simulink model "Terasic_Simscape_LQR_2PWM_DISTURBED"  (R2024b)
settings: Solver=VariableStepAuto  StartTime=0.0  StopTime=40  RelTol=1e-3  AbsTol=1e-3  EnableMultiTasking=on
undefined symbols (not defined in the file or in its folder): chassis_mass, dt, gear, joint_friction, K_dlqr, k_t, max_pwm, motor_max_torque, R_int, rotor_inertia, V_nom, wheel_mass, wheel_radius, wheel_track, X, Y, Z
libraries: sm_lib x29, nesl_utility x18, simulink x2
settings Model: Creator=monet  LastModifiedBy=monet
settings SolverCC: AutoScaleAbsTol=off  AlgebraicLoopSolver=TrustRegion  MaxZcPerStep=1
settings DataIOCC: LimitDataPoints=on  MaxDataPoints=10000
settings OptimizationCC: BlockReduction=off  DefaultParameterBehavior=Inlined  BufferReuse=off  ReuseModelBlockBuffer=off  LifeSpan=inf
settings DebuggingCC: UnconnectedInputMsg=warning  UnconnectedOutputMsg=warning  UnconnectedLineMsg=warning  AllowSymbolicDim=off  SubsystemReferenceDiagnosticForUnitTest=warning  SFUnexpectedBacktrackingDiag=warning  SFNoUnconditionalDefaultTransitionDiag=warning  SFExecutionAtInitializationDiag=none  ArithmeticOperatorsInVariantConditions=warning
settings ModelReferenceCC: EnableRefExpFcnMdlSchedulingChecks=on
settings SFSimCC: SimUseLocalCustomCode=off  CustomCodeUndefinedFunction=UseInterfaceOnly
settings RTWCC: RTWUseLocalCustomCode=off  GPUComputeCapability=3.5  DLArmComputeVersion=19.05
settings CodeAppCC: StateflowObjectComments=on
settings GRTTargetCC: TargetLangStandard=C89/C90 (ANSI)
settings ConfigComp: CovMetricSettings=dw  CovSaveCumulativeToWorkspaceVar=on  CovSaveSingleToWorkspaceVar=on  CovExternalEMLEnable=off  CovSFcnEnable=off
settings SimscapeCC: SimscapeLogType=all  SimscapeLogSimulationStatistics=on  SimscapeLogDataHistory=10000
settings ExplorerConfigSet: InternalSimMechanicsExplorerSettings="<ExplorerConfiguration><canonicalview>default</canonicalview><AnimationSetting><BasePlaybackSpeed>1.0</BasePlaybackSpeed><PlaybackSpeedFactor>1.0</PlaybackSpeedFactor></AnimationSetting><TilePanel><TileInfo><Tiles Columns=\"1\" Count=\"1\" Rows=\"1\"><Column Weight=\"1\"/><Row Weight=\"1\"/><Tile Height=\"1\" Width=\"1\" X=\"0\" Y=\"0\"/></Tiles></TileInfo><SceneInfo><SceneViewer><BGColor><R>0.60000002384185791</R><G>0.60000002384185791</G><B>0.60000002384185791</B></BGColor><Camera><DoPerspective>off</DoPerspective><Position><X>0.347323457562067783</X><Y>0.515589851628267981</Y><Z>1.53123320149964282</Z></Position><Center><X>0.0533393895155996889</X><Y>-0.0401565567814901048</Y><Z>0.259834581816526411</Z></Center><Up><X>0.974608991684094539</X><Y>-0.00336145818059463419</Y><Z>-0.22388839614283837</Z></Up><ViewLimDist>1</ViewLimDist><YLim>0.251495735782762964</YLim><XLim>0.488937298095312722</XLim></Camera></SceneViewer></SceneInfo></TilePanel><MechEditorPanel><Cameras/><GfxPanelCameraMap/><VideoCreator><PlaybackSpeedRatio>1.0</PlaybackSpeedRatio><FrameRate>30</FrameRate><VideoFormat>Motion JPEG AVI</VideoFormat><FrameSize>auto</FrameSize></VideoCreator></MechEditorPanel></ExplorerConfiguration>"

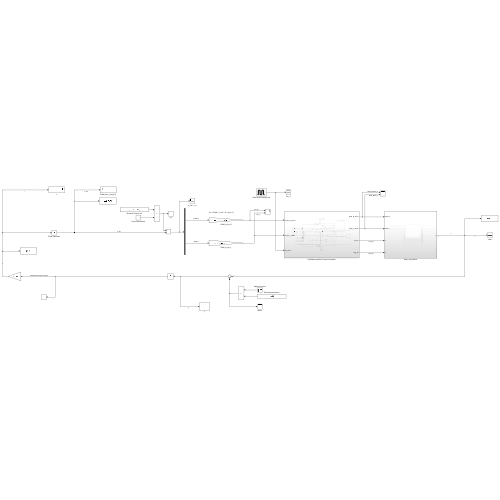
[thumbnail: Simulink's stored preview of the top-level diagram]
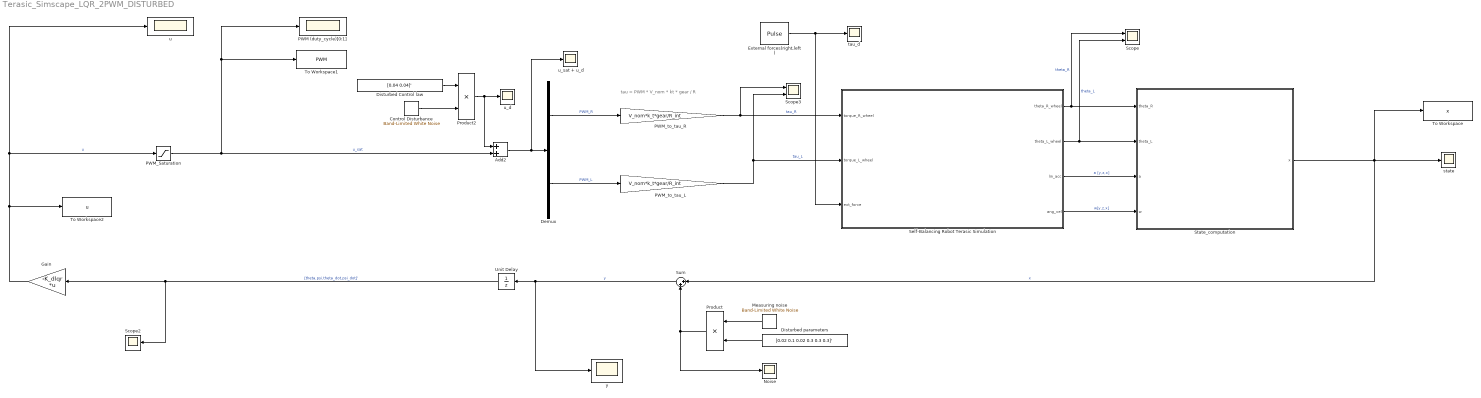
== system Terasic_Simscape_LQR_2PWM_DISTURBED ==
  note: tau = PWM * V_nom * kt * gear / R
  Add2 : Sum
  Control Disturbance : simulink/Sources/Band-Limited White Noise  Cov=[0.001]  Ts=0.1  seed=[23341]
  Demux : Demux  Outputs=2
  Disturbed Control law : Constant  Value=[0.04 0.04]'
  Disturbed parameters : Constant  Value=[0.02 0.1 0.02 0.3 0.3 0.3]'
  External forces(right,left) : DiscretePulseGenerator  PulseType=Time based  Amplitude=0.5  Period=5  PulseWidth=10  PhaseDelay=2
  Gain : Gain  Gain=-K_dlqr  Multiplication=Matrix(K*u)
  Measuring noise : simulink/Sources/Band-Limited White Noise  Cov=[0.001]  Ts=0.1  seed=[23341]
  Noise : Scope
  PWM (duty_cycle)[0:1] : Scope
  PWM_Saturation : Saturate  UpperLimit=max_pwm  LowerLimit=-max_pwm
  PWM_to_tau_L : Gain  Gain=V_nom*k_t*gear/R_int
  PWM_to_tau_R : Gain  Gain=V_nom*k_t*gear/R_int
  Product : Product
  Product2 : Product
  Scope : Scope  NumInputPorts=2
  Scope2 : Scope
  Scope3 : Scope  NumInputPorts=2
  Self-Balancing Robot Terasic Simulation : Subsystem
  State_computation : Subsystem
  Sum : Sum  Inputs=|++
  To Workspace : ToWorkspace  VariableName=x  SaveFormat=Timeseries  SampleTime=-1
  To Workspace1 : ToWorkspace  VariableName=PWM  SaveFormat=Timeseries  SampleTime=-1
  To Workspace2 : ToWorkspace  VariableName=u  SaveFormat=Timeseries  SampleTime=-1
  Unit Delay : UnitDelay  InitialCondition=[0;0;0;0;0;0]  SampleTime=dt  HasFrameUpgradeWarning=on
  state : Scope
  tau_d : Scope
  u : Scope
  u_d : Scope
  u_sat + u_d : Scope
  y : Scope
  wires:
  PWM_to_tau_L/1 -> Self-Balancing Robot Terasic Simulation/2(torque_L_wheel), Scope3/2  "tau_L"
  PWM_to_tau_R/1 -> Self-Balancing Robot Terasic Simulation/1(torque_R_wheel), Scope3/1  "tau_R"
  PWM_Saturation/1 -> To Workspace1/1, PWM (duty_cycle)[0:1]/1, Add2/2  "u_sat"
  Demux/1 -> PWM_to_tau_R/1  "PWM_R"
  Demux/2 -> PWM_to_tau_L/1  "PWM_L"
  Unit Delay/1 -> Scope2/1, Gain/1  "[theta,psi,theta_dot,psi_dot]'"
  Gain/1 -> u/1, PWM_Saturation/1, To Workspace2/1  "u"
  State_computation/1(x) -> Sum/1, To Workspace/1, state/1  "x"
  Self-Balancing Robot Terasic Simulation/2(theta_L_wheel) -> State_computation/2(theta_L), Scope/2  "theta_L"
  Self-Balancing Robot Terasic Simulation/1(theta_R_wheel) -> State_computation/1(theta_R), Scope/1  "theta_R"
  Self-Balancing Robot Terasic Simulation/4(ang_vel) -> State_computation/4(w)  "w[y,z,x]"
  Self-Balancing Robot Terasic Simulation/3(lin_acc) -> State_computation/3(a)  "a [y,z,x]"
  Control Disturbance/1 -> Product2/2
  Product2/1 -> u_d/1, Add2/1
  Disturbed Control law/1 -> Product2/1
  External forces(right,left)/1 -> Self-Balancing Robot Terasic Simulation/3(ext_force), tau_d/1
  Sum/1 -> y/1, Unit Delay/1  "y"
  Measuring noise/1 -> Product/1
  Disturbed parameters/1 -> Product/2
  Product/1 -> Noise/1, Sum/2
  Add2/1 -> u_sat + u_d/1, Demux/1

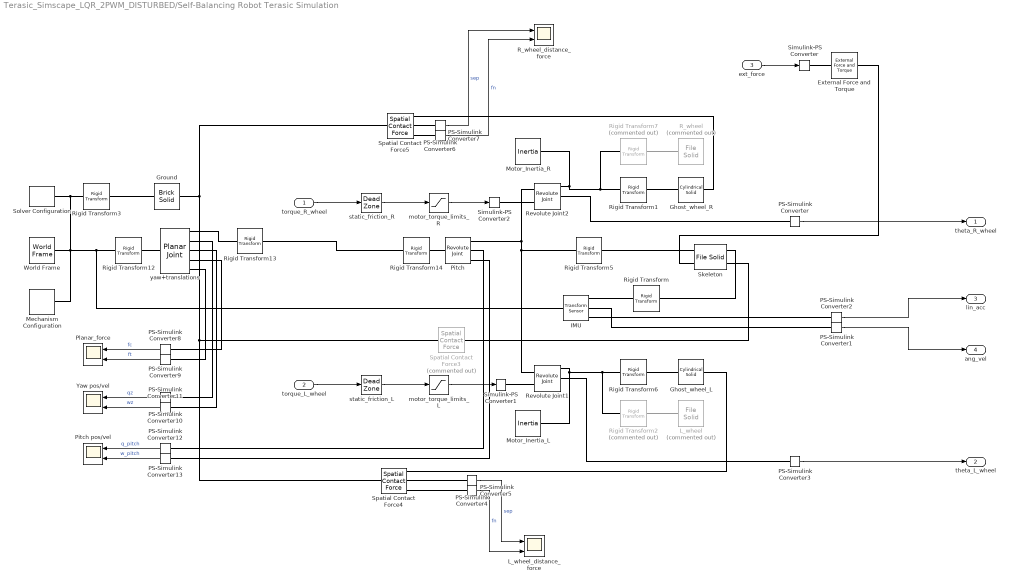
== system Terasic_Simscape_LQR_2PWM_DISTURBED/Self-Balancing Robot Terasic Simulation ==
  torque_R_wheel : Inport
  torque_L_wheel : Inport  Port=2
  ext_force : Inport  Port=3
  External Force and Torque : sm_lib/Forces and Torques/External Force and Torque  EnableForceX=off  EnableForceY=on  EnableForceZ=off  EnableForce=off  ForceResolutionFrame=AttachedFrame  EnableTorqueX=off  EnableTorqueY=off  EnableTorqueZ=off  EnableTorque=off  TorqueResolutionFrame=AttachedFrame
  Ghost_wheel_L : sm_lib/Body Elements/Cylindrical Solid  CylinderRadius=wheel_radius  CylinderRadiusUnits=m  CylinderLength=wheel_thickness  CylinderLengthUnits=m  ExportEntireGeometry=on  InertiaType=CalculateFromGeometry  BasedOnType=Mass  Density=1000  DensityUnits=kg/m^3  Mass=wheel_mass  MassUnits=kg  CenterOfMass=[0 0 0]  CenterOfMassUnits=m  MomentsOfInertia=[1 1 1]  MomentsOfInertiaUnits=kg*m^2  ProductsOfInertia=[0 0 0]  ProductsOfInertiaUnits=kg*m^2  GraphicType=FromGeometry  MarkerShape=Sphere  MarkerSize=10  GraphicVisPropType=SimpleVisualProperties  GraphicDiffuseColor=[1 0 0]  GraphicOpacity=0.1  GraphicSpecularColor=[0.5 0.5 0.5 1.0]  GraphicAmbientColor=[0.15 0.15 0.15 1.0]  GraphicEmissiveColor=[0.0 0.0 0.0 1.0]  GraphicShininess=75  DoExposeReferenceFrame=off  SerializedFrames=<Frames><Frame><Id>Frame1</Id><Value><Name>F1</Name><Origin><Source>ReferenceFrame</Source><FeatureName></FeatureName></Origin><PrimaryAxis><DefinedDirection>+Z</DefinedDirection><Source>ReferenceFrame</Source><SourceDirection>+Z</SourceDirection><FeatureName></FeatureName></PrimaryAxis><SecondaryAxis><DefinedDirection>+X</DefinedDirection><Source>ReferenceFrame</Source><SourceDirection>+X</SourceDirection><FeatureName></FeatureName></SecondaryAxis></Value></Frame></Frames>
  Ghost_wheel_R : sm_lib/Body Elements/Cylindrical Solid  CylinderRadius=wheel_radius  CylinderRadiusUnits=m  CylinderLength=wheel_thickness  CylinderLengthUnits=m  ExportEntireGeometry=on  InertiaType=CalculateFromGeometry  BasedOnType=Mass  Density=1000  DensityUnits=kg/m^3  Mass=wheel_mass  MassUnits=kg  CenterOfMass=[0 0 0]  CenterOfMassUnits=m  MomentsOfInertia=[1 1 1]  MomentsOfInertiaUnits=kg*m^2  ProductsOfInertia=[0 0 0]  ProductsOfInertiaUnits=kg*m^2  GraphicType=FromGeometry  MarkerShape=Sphere  MarkerSize=10  GraphicVisPropType=SimpleVisualProperties  GraphicDiffuseColor=[1 0 0]  GraphicOpacity=0.1  GraphicSpecularColor=[0.5 0.5 0.5 1.0]  GraphicAmbientColor=[0.15 0.15 0.15 1.0]  GraphicEmissiveColor=[0.0 0.0 0.0 1.0]  GraphicShininess=75  DoExposeReferenceFrame=off  SerializedFrames=<Frames><Frame><Id>Frame1</Id><Value><Name>F1</Name><Origin><Source>ReferenceFrame</Source><FeatureName></FeatureName></Origin><PrimaryAxis><DefinedDirection>+Z</DefinedDirection><Source>ReferenceFrame</Source><SourceDirection>+Z</SourceDirection><FeatureName></FeatureName></PrimaryAxis><SecondaryAxis><DefinedDirection>+X</DefinedDirection><Source>ReferenceFrame</Source><SourceDirection>+X</SourceDirection><FeatureName></FeatureName></SecondaryAxis></Value></Frame></Frames>
  Ground : sm_lib/Body Elements/Brick Solid  BrickDimensions=[2 2 0.003]  BrickDimensionsUnits=m  ExportEntireGeometry=on  InertiaType=CalculateFromGeometry  BasedOnType=Density  Density=1000  DensityUnits=kg/m^3  Mass=1  MassUnits=kg  CenterOfMass=[0 0 0]  CenterOfMassUnits=m  MomentsOfInertia=[1 1 1]  MomentsOfInertiaUnits=kg*m^2  ProductsOfInertia=[0 0 0]  ProductsOfInertiaUnits=kg*m^2  GraphicType=FromGeometry  MarkerShape=Sphere  MarkerSize=10  GraphicVisPropType=SimpleVisualProperties  GraphicDiffuseColor=[0.9412 0.9412 0.9412]  GraphicOpacity=1  GraphicSpecularColor=[0.5 0.5 0.5 1.0]  GraphicAmbientColor=[0.15 0.15 0.15 1.0]  GraphicEmissiveColor=[0.0 0.0 0.0 1.0]  GraphicShininess=75  DoExposeReferenceFrame=on  SerializedFrames=<Frames/>
  IMU : sm_lib/Frames and Transforms/Transform Sensor  MeasurementFrame=Follower  RotationSequence=XYX  SenseAngle=off  SenseAxis=off  SenseQ=off  SenseR=off  SenseRotationSequence=off  SenseOmegaX=off  SenseOmegaY=off  SenseOmegaZ=off  SenseOmega=on  SenseQDot=off  SenseRDot=off  SenseRotationSequenceDot=off  SenseAlphaX=off  SenseAlphaY=off  SenseAlphaZ=off  SenseAlpha=off  SenseQDDot=off  SenseRDDot=off  SenseX=off  SenseY=off  SenseZ=off  SenseXYZ=off  SenseRad=off  SenseAzim=off  SenseDist=off  SenseInc=off  SenseXDot=off  SenseYDot=off  SenseZDot=off  SenseXYZDot=off  SenseRadDot=off  SenseAzimDot=off  SenseDistDot=off  SenseIncDot=off  SenseXDDot=off  SenseYDDot=off  SenseZDDot=off  SenseXYZDDot=on  SenseRadDDot=off  SenseAzimDDot=off  SenseDistDDot=off  SenseIncDDot=off
  L_wheel : sm_lib/Body Elements/File Solid  Commented=on  ExtGeomFileName=C:\Users\monet\Documents\UNIVERSITA'\MAGISTRALE\Tirocinio_University_of_Poznan\MuJoco&Simscape\STL_NEW - Copia\wheel_complete_simulation.STL  UnitType=Custom  ExtGeomFileUnits=m  StepReaderType=HEX  ExportConvexHullGeometry=on  InertiaType=CalculateFromGeometry  BasedOnType=Mass  Density=1000  DensityUnits=kg/m^3  Mass=1e-6  MassUnits=kg  CenterOfMass=[0 0 0]  CenterOfMassUnits=m  MomentsOfInertia=[1 1 1]  MomentsOfInertiaUnits=kg*m^2  ProductsOfInertia=[0 0 0]  ProductsOfInertiaUnits=kg*m^2  GraphicType=FromGeometry  MarkerShape=Sphere  MarkerSize=10  GraphicVisPropType=SimpleVisualProperties  GraphicDiffuseColor=[0.6353 0.07843 0.1843]  GraphicOpacity=1  GraphicSpecularColor=[0.5 0.5 0.5 1.0]  GraphicAmbientColor=[0.15 0.15 0.15 1.0]  GraphicEmissiveColor=[0.0 0.0 0.0 1.0]  GraphicShininess=75  DoExposeReferenceFrame=off  SerializedFrames=<Frames><Frame><Id>Frame1</Id><Value><Name>F1</Name><Origin><Source>ReferenceFrame</Source><FeatureName></FeatureName></Origin><PrimaryAxis><DefinedDirection>+Z</DefinedDirection><Source>ReferenceFrame</Source><SourceDirection>+Z</SourceDirection><FeatureName></FeatureName></PrimaryAxis><SecondaryAxis><DefinedDirection>+X</DefinedDirection><Source>ReferenceFrame</Source><SourceDirection>+X</SourceDirection><FeatureName></FeatureName></SecondaryAxis></Value></Frame></Frames>
  L_wheel_distance_force : Scope  NumInputPorts=2
  Mechanism Configuration : sm_lib/Utilities/Mechanism Configuration  UniformGravity=Constant  GravityVector=[-9.81 0 0]  GravityVectorUnits=m/s^2  LinearizationDelta=0.001  JointModeTransitionNonlinearIterations=2
  Motor_Inertia_L : sm_lib/Body Elements/Inertia  InertiaType=Custom  Mass=1e-6  MassUnits=kg  CenterOfMass=[0 0 0]  CenterOfMassUnits=m  MomentsOfInertia=[0 0 rotor_inertia]  MomentsOfInertiaUnits=kg*m^2  ProductsOfInertia=[0 0 0]  ProductsOfInertiaUnits=kg*m^2  GraphicType=Marker  MarkerShape=Inertia  MarkerSize=20  GraphicVisPropType=SimpleVisualProperties  GraphicDiffuseColor=[0.5 0.5 0.5]  GraphicOpacity=1  GraphicSpecularColor=[0.5 0.5 0.5 1.0]  GraphicAmbientColor=[0.15 0.15 0.15 1.0]  GraphicEmissiveColor=[0.0 0.0 0.0 1.0]  GraphicShininess=75
  Motor_Inertia_R : sm_lib/Body Elements/Inertia  InertiaType=Custom  Mass=1e-6  MassUnits=kg  CenterOfMass=[0 0 0]  CenterOfMassUnits=m  MomentsOfInertia=[0 0 rotor_inertia]  MomentsOfInertiaUnits=kg*m^2  ProductsOfInertia=[0 0 0]  ProductsOfInertiaUnits=kg*m^2  GraphicType=Marker  MarkerShape=Inertia  MarkerSize=20  GraphicVisPropType=SimpleVisualProperties  GraphicDiffuseColor=[0.5 0.5 0.5]  GraphicOpacity=1  GraphicSpecularColor=[0.5 0.5 0.5 1.0]  GraphicAmbientColor=[0.15 0.15 0.15 1.0]  GraphicEmissiveColor=[0.0 0.0 0.0 1.0]  GraphicShininess=75
  PS-Simulink Converter{,1..13} (14 alike) : nesl_utility/PS-Simulink Converter  PhysicalDomain=network_engine_domain  SubClassName=ps_output  LeftPortType=input  RightPortType=output  PseudoPeriodic=off  Frequencies=[]  VectorFormat=inherit  Unit=inherit  AffineConversion=off
  Pitch : sm_lib/Joints/Revolute Joint  JointMode=Normal  CompositeWrenchDir=FollowerOnBase  CompositeWrenchFrame=BaseFrame  SenseConstraintForce=off  SenseConstraintTorque=off  SenseTotalForce=off  SenseTotalTorque=off  PositionTargetSpecify=off  PositionTargetPriority=High  PositionTargetValue=0  PositionTargetValueUnits=deg  VelocityTargetSpecify=off  VelocityTargetPriority=High  VelocityTargetValue=0  VelocityTargetValueUnits=deg/s  EquilibriumPosition=0  EquilibriumPositionUnits=deg  SpringStiffness=0  SpringStiffnessUnits=N*m/deg  DampingCoefficient=0  DampingCoefficientUnits=N*m/(deg/s)  LowerLimitSpecify=off  LowerLimitBound=-90  LowerLimitBoundUnits=deg  LowerLimitStiffness=1e4  LowerLimitStiffnessUnits=N*m/deg  LowerLimitDamping=10  LowerLimitDampingUnits=N*m/(deg/s)  LowerLimitTransitionRegionWidth=0.1  LowerLimitTransitionRegionWidthUnits=deg  UpperLimitSpecify=off  UpperLimitBound=90  UpperLimitBoundUnits=deg  UpperLimitStiffness=1e4  UpperLimitStiffnessUnits=N*m/deg  UpperLimitDamping=10  UpperLimitDampingUnits=N*m/(deg/s)  UpperLimitTransitionRegionWidth=0.1  UpperLimitTransitionRegionWidthUnits=deg  TorqueActuationMode=NoTorque  MotionActuationMode=ComputedMotion  SensePosition=on  SenseVelocity=on  SenseAcceleration=off  SenseTorqueForce=off  SenseLowerLimitTorqueForce=off  SenseUpperLimitTorqueForce=off
  Pitch pos/vel : Scope  NumInputPorts=2
  Planar_force : Scope  NumInputPorts=2
  R_wheel : sm_lib/Body Elements/File Solid  Commented=on  ExtGeomFileName=C:\Users\monet\Documents\UNIVERSITA'\MAGISTRALE\Tirocinio_University_of_Poznan\MuJoco&Simscape\STL_NEW - Copia\wheel_complete_simulation.STL  UnitType=Custom  ExtGeomFileUnits=m  StepReaderType=HEX  ExportConvexHullGeometry=on  InertiaType=CalculateFromGeometry  BasedOnType=Mass  Density=1000  DensityUnits=kg/m^3  Mass=1e-6  MassUnits=kg  CenterOfMass=[0 0 0]  CenterOfMassUnits=m  MomentsOfInertia=[1 1 1]  MomentsOfInertiaUnits=kg*m^2  ProductsOfInertia=[0 0 0]  ProductsOfInertiaUnits=kg*m^2  GraphicType=FromGeometry  MarkerShape=Sphere  MarkerSize=10  GraphicVisPropType=SimpleVisualProperties  GraphicDiffuseColor=[0.6353 0.07843 0.1843]  GraphicOpacity=1  GraphicSpecularColor=[0.5 0.5 0.5 1.0]  GraphicAmbientColor=[0.15 0.15 0.15 1.0]  GraphicEmissiveColor=[0.0 0.0 0.0 1.0]  GraphicShininess=75  DoExposeReferenceFrame=off  SerializedFrames=<Frames><Frame><Id>Frame1</Id><Value><Name>F1</Name><Origin><Source>ReferenceFrame</Source><FeatureName></FeatureName></Origin><PrimaryAxis><DefinedDirection>+Z</DefinedDirection><Source>ReferenceFrame</Source><SourceDirection>+Z</SourceDirection><FeatureName></FeatureName></PrimaryAxis><SecondaryAxis><DefinedDirection>+X</DefinedDirection><Source>ReferenceFrame</Source><SourceDirection>+X</SourceDirection><FeatureName></FeatureName></SecondaryAxis></Value></Frame></Frames>
  R_wheel_distance_force : Scope  NumInputPorts=2
  Revolute Joint1 : sm_lib/Joints/Revolute Joint  JointMode=Normal  CompositeWrenchDir=FollowerOnBase  CompositeWrenchFrame=BaseFrame  SenseConstraintForce=off  SenseConstraintTorque=off  SenseTotalForce=off  SenseTotalTorque=off  PositionTargetSpecify=off  PositionTargetPriority=High  PositionTargetValue=0  PositionTargetValueUnits=deg  VelocityTargetSpecify=off  VelocityTargetPriority=High  VelocityTargetValue=0  VelocityTargetValueUnits=deg/s  EquilibriumPosition=0  EquilibriumPositionUnits=deg  SpringStiffness=0  SpringStiffnessUnits=N*m/deg  DampingCoefficient=joint_damping  DampingCoefficientUnits=N*m*s/rad  LowerLimitSpecify=off  LowerLimitBound=-90  LowerLimitBoundUnits=deg  LowerLimitStiffness=1e4  LowerLimitStiffnessUnits=N*m/deg  LowerLimitDamping=10  LowerLimitDampingUnits=N*m/(deg/s)  LowerLimitTransitionRegionWidth=0.1  LowerLimitTransitionRegionWidthUnits=deg  UpperLimitSpecify=off  UpperLimitBound=90  UpperLimitBoundUnits=deg  UpperLimitStiffness=1e4  UpperLimitStiffnessUnits=N*m/deg  UpperLimitDamping=10  UpperLimitDampingUnits=N*m/(deg/s)  UpperLimitTransitionRegionWidth=0.1  UpperLimitTransitionRegionWidthUnits=deg  TorqueActuationMode=InputTorque  MotionActuationMode=ComputedMotion  SensePosition=on  SenseVelocity=on  SenseAcceleration=off  SenseTorqueForce=off  SenseLowerLimitTorqueForce=off  SenseUpperLimitTorqueForce=off
  Revolute Joint2 : sm_lib/Joints/Revolute Joint  JointMode=Normal  CompositeWrenchDir=FollowerOnBase  CompositeWrenchFrame=BaseFrame  SenseConstraintForce=off  SenseConstraintTorque=off  SenseTotalForce=off  SenseTotalTorque=off  PositionTargetSpecify=off  PositionTargetPriority=High  PositionTargetValue=0  PositionTargetValueUnits=deg  VelocityTargetSpecify=off  VelocityTargetPriority=High  VelocityTargetValue=0  VelocityTargetValueUnits=deg/s  EquilibriumPosition=0  EquilibriumPositionUnits=deg  SpringStiffness=0  SpringStiffnessUnits=N*m/deg  DampingCoefficient=joint_damping  DampingCoefficientUnits=N*m*s/rad  LowerLimitSpecify=off  LowerLimitBound=-90  LowerLimitBoundUnits=deg  LowerLimitStiffness=1e4  LowerLimitStiffnessUnits=N*m/deg  LowerLimitDamping=10  LowerLimitDampingUnits=N*m/(deg/s)  LowerLimitTransitionRegionWidth=0.1  LowerLimitTransitionRegionWidthUnits=deg  UpperLimitSpecify=off  UpperLimitBound=90  UpperLimitBoundUnits=deg  UpperLimitStiffness=1e4  UpperLimitStiffnessUnits=N*m/deg  UpperLimitDamping=10  UpperLimitDampingUnits=N*m/(deg/s)  UpperLimitTransitionRegionWidth=0.1  UpperLimitTransitionRegionWidthUnits=deg  TorqueActuationMode=InputTorque  MotionActuationMode=ComputedMotion  SensePosition=on  SenseVelocity=on  SenseAcceleration=off  SenseTorqueForce=off  SenseLowerLimitTorqueForce=off  SenseUpperLimitTorqueForce=off
  Rigid Transform : sm_lib/Frames and Transforms/Rigid Transform  RotationMethod=None  FollAlignAxisA=+X  BaseAlignAxisA=+Y  FollAlignAxisB=+Y  BaseAlignAxisB=+Z  RotationStandardAxis=+Z  RotationAngle=0  RotationAngleUnits=deg  RotationArbitraryAxis=[0 0 1]  RotationSequenceAxes=FollowerAxes  RotationSequence=XYX  RotationSequenceAngles=[0 0 0]  RotationSequenceAnglesUnits=deg  RotationMatrix=[1 0 0;0 1 0;0 0 1]  Quaternion=[1 0 0 0]  TranslationMethod=Cartesian  TranslationCartesianOffset=[20 20 -85]  TranslationCartesianOffsetUnits=mm  TranslationStandardAxis=+Z  TranslationStandardOffset=0  TranslationStandardOffsetUnits=m  TranslationROffset=0  TranslationROffsetUnits=m  TranslationThetaOffset=0  TranslationThetaOffsetUnits=deg  TranslationZOffset=0  TranslationZOffsetUnits=m
  Rigid Transform1 : sm_lib/Frames and Transforms/Rigid Transform  RotationMethod=RotationSequence  FollAlignAxisA=+X  BaseAlignAxisA=+Y  FollAlignAxisB=+Y  BaseAlignAxisB=+Z  RotationStandardAxis=+Z  RotationAngle=0  RotationAngleUnits=deg  RotationArbitraryAxis=[0 0 1]  RotationSequenceAxes=FollowerAxes  RotationSequence=XYX  RotationSequenceAngles=[0 0 0]  RotationSequenceAnglesUnits=deg  RotationMatrix=[-1 0 0;0 -1 0;0 0 1]  Quaternion=[1 0 0 0]  TranslationMethod=Cartesian  TranslationCartesianOffset=[0 0 82]  TranslationCartesianOffsetUnits=mm  TranslationStandardAxis=+Z  TranslationStandardOffset=0  TranslationStandardOffsetUnits=m  TranslationROffset=0  TranslationROffsetUnits=m  TranslationThetaOffset=0  TranslationThetaOffsetUnits=deg  TranslationZOffset=0  TranslationZOffsetUnits=m
  Rigid Transform12 : sm_lib/Frames and Transforms/Rigid Transform  RotationMethod=RotationSequence  FollAlignAxisA=+X  BaseAlignAxisA=+Y  FollAlignAxisB=+Y  BaseAlignAxisB=+Z  RotationStandardAxis=+Z  RotationAngle=0  RotationAngleUnits=deg  RotationArbitraryAxis=[0 0 1]  RotationSequenceAxes=FollowerAxes  RotationSequence=XYX  RotationSequenceAngles=[0 90 0]  RotationSequenceAnglesUnits=deg  RotationMatrix=[1 0 0;0 1 0;0 0 1]  Quaternion=[1 0 0 0]  TranslationMethod=Cartesian  TranslationCartesianOffset=[0.032+0.002949/2 0 0]  TranslationCartesianOffsetUnits=m  TranslationStandardAxis=+Z  TranslationStandardOffset=0  TranslationStandardOffsetUnits=m  TranslationROffset=0  TranslationROffsetUnits=m  TranslationThetaOffset=0  TranslationThetaOffsetUnits=deg  TranslationZOffset=0  TranslationZOffsetUnits=m
  Rigid Transform13 : sm_lib/Frames and Transforms/Rigid Transform  RotationMethod=RotationSequence  FollAlignAxisA=+X  BaseAlignAxisA=+Y  FollAlignAxisB=+Y  BaseAlignAxisB=+Z  RotationStandardAxis=+Z  RotationAngle=0  RotationAngleUnits=deg  RotationArbitraryAxis=[0 0 1]  RotationSequenceAxes=FollowerAxes  RotationSequence=XYX  RotationSequenceAngles=[0 -90 0]  RotationSequenceAnglesUnits=deg  RotationMatrix=[1 0 0;0 1 0;0 0 1]  Quaternion=[1 0 0 0]  TranslationMethod=Cartesian  TranslationCartesianOffset=[0 0 0]  TranslationCartesianOffsetUnits=m  TranslationStandardAxis=+Z  TranslationStandardOffset=0  TranslationStandardOffsetUnits=m  TranslationROffset=0  TranslationROffsetUnits=m  TranslationThetaOffset=0  TranslationThetaOffsetUnits=deg  TranslationZOffset=0  TranslationZOffsetUnits=m
  Rigid Transform14 : sm_lib/Frames and Transforms/Rigid Transform  RotationMethod=RotationSequence  FollAlignAxisA=+X  BaseAlignAxisA=+Y  FollAlignAxisB=+Y  BaseAlignAxisB=+Z  RotationStandardAxis=+Z  RotationAngle=0  RotationAngleUnits=deg  RotationArbitraryAxis=[0 0 1]  RotationSequenceAxes=FollowerAxes  RotationSequence=XYX  RotationSequenceAngles=[90 0 0]  RotationSequenceAnglesUnits=deg  RotationMatrix=[1 0 0;0 1 0;0 0 1]  Quaternion=[1 0 0 0]  TranslationMethod=Cartesian  TranslationCartesianOffset=[0 0 0]  TranslationCartesianOffsetUnits=m  TranslationStandardAxis=+Z  TranslationStandardOffset=0  TranslationStandardOffsetUnits=m  TranslationROffset=0  TranslationROffsetUnits=m  TranslationThetaOffset=0  TranslationThetaOffsetUnits=deg  TranslationZOffset=0  TranslationZOffsetUnits=m
  Rigid Transform2 : sm_lib/Frames and Transforms/Rigid Transform  Commented=on  RotationMethod=RotationSequence  FollAlignAxisA=+X  BaseAlignAxisA=+Y  FollAlignAxisB=+Y  BaseAlignAxisB=+Z  RotationStandardAxis=+Z  RotationAngle=0  RotationAngleUnits=deg  RotationArbitraryAxis=[0 0 1]  RotationSequenceAxes=FollowerAxes  RotationSequence=XYX  RotationSequenceAngles=[180 90 0]  RotationSequenceAnglesUnits=deg  RotationMatrix=[1 0 0;0 1 0;0 0 1]  Quaternion=[1 0 0 0]  TranslationMethod=Cartesian  TranslationCartesianOffset=[0 0 -82]  TranslationCartesianOffsetUnits=mm  TranslationStandardAxis=+Z  TranslationStandardOffset=0  TranslationStandardOffsetUnits=m  TranslationROffset=0  TranslationROffsetUnits=m  TranslationThetaOffset=0  TranslationThetaOffsetUnits=deg  TranslationZOffset=0  TranslationZOffsetUnits=m
  Rigid Transform3 : sm_lib/Frames and Transforms/Rigid Transform  RotationMethod=RotationSequence  FollAlignAxisA=+X  BaseAlignAxisA=+Y  FollAlignAxisB=+Y  BaseAlignAxisB=+Z  RotationStandardAxis=+Z  RotationAngle=0  RotationAngleUnits=deg  RotationArbitraryAxis=[0 0 1]  RotationSequenceAxes=FollowerAxes  RotationSequence=XYX  RotationSequenceAngles=[0 90 0]  RotationSequenceAnglesUnits=deg  RotationMatrix=[1 0 0;0 1 0;0 0 1]  Quaternion=[1 0 0 0]  TranslationMethod=None  TranslationCartesianOffset=[0 0 0]  TranslationCartesianOffsetUnits=m  TranslationStandardAxis=+Z  TranslationStandardOffset=0  TranslationStandardOffsetUnits=m  TranslationROffset=0  TranslationROffsetUnits=m  TranslationThetaOffset=0  TranslationThetaOffsetUnits=deg  TranslationZOffset=0  TranslationZOffsetUnits=m
  Rigid Transform5 : sm_lib/Frames and Transforms/Rigid Transform  RotationMethod=RotationSequence  FollAlignAxisA=+X  BaseAlignAxisA=+Y  FollAlignAxisB=+Y  BaseAlignAxisB=+Z  RotationStandardAxis=+Z  RotationAngle=0  RotationAngleUnits=deg  RotationArbitraryAxis=[0 0 1]  RotationSequenceAxes=FollowerAxes  RotationSequence=XYX  RotationSequenceAngles=[0 90 0]  RotationSequenceAnglesUnits=deg  RotationMatrix=[1 0 0;0 1 0;0 0 1]  Quaternion=[1 0 0 0]  TranslationMethod=None  TranslationCartesianOffset=[0 0 0]  TranslationCartesianOffsetUnits=m  TranslationStandardAxis=+Z  TranslationStandardOffset=0  TranslationStandardOffsetUnits=m  TranslationROffset=0  TranslationROffsetUnits=m  TranslationThetaOffset=0  TranslationThetaOffsetUnits=deg  TranslationZOffset=0  TranslationZOffsetUnits=m
  Rigid Transform6 : sm_lib/Frames and Transforms/Rigid Transform  RotationMethod=RotationSequence  FollAlignAxisA=+X  BaseAlignAxisA=+Y  FollAlignAxisB=+Y  BaseAlignAxisB=+Z  RotationStandardAxis=+Z  RotationAngle=0  RotationAngleUnits=deg  RotationArbitraryAxis=[0 0 1]  RotationSequenceAxes=FollowerAxes  RotationSequence=XYX  RotationSequenceAngles=[180 0 0]  RotationSequenceAnglesUnits=deg  RotationMatrix=[1 0 0;0 1 0;0 0 1]  Quaternion=[1 0 0 0]  TranslationMethod=Cartesian  TranslationCartesianOffset=[0 0 -82]  TranslationCartesianOffsetUnits=mm  TranslationStandardAxis=+Z  TranslationStandardOffset=0  TranslationStandardOffsetUnits=m  TranslationROffset=0  TranslationROffsetUnits=m  TranslationThetaOffset=0  TranslationThetaOffsetUnits=deg  TranslationZOffset=0  TranslationZOffsetUnits=m
  Rigid Transform7 : sm_lib/Frames and Transforms/Rigid Transform  Commented=on  RotationMethod=RotationSequence  FollAlignAxisA=+X  BaseAlignAxisA=+Y  FollAlignAxisB=+Y  BaseAlignAxisB=+Z  RotationStandardAxis=+Z  RotationAngle=0  RotationAngleUnits=deg  RotationArbitraryAxis=[0 0 1]  RotationSequenceAxes=FollowerAxes  RotationSequence=XYX  RotationSequenceAngles=[0 90 0]  RotationSequenceAnglesUnits=deg  RotationMatrix=[-1 0 0;0 -1 0;0 0 1]  Quaternion=[1 0 0 0]  TranslationMethod=Cartesian  TranslationCartesianOffset=[0 0 82]  TranslationCartesianOffsetUnits=mm  TranslationStandardAxis=+Z  TranslationStandardOffset=0  TranslationStandardOffsetUnits=m  TranslationROffset=0  TranslationROffsetUnits=m  TranslationThetaOffset=0  TranslationThetaOffsetUnits=deg  TranslationZOffset=0  TranslationZOffsetUnits=m
  Simulink-PS Converter : nesl_utility/Simulink-PS Converter  PhysicalDomain=network_engine_domain  SubClassName=ps_input  LeftPortType=input  RightPortType=output  PseudoPeriodic=off  Frequencies=[]  NoiseDistribution=none  NoiseParameters=[]  Unit=1  AffineConversion=off  FilteringAndDerivatives=provide  SimscapeFilterOrder=1  InputFilterTimeConstant=0.001  UdotUserProvided=0
  Simulink-PS Converter1 : nesl_utility/Simulink-PS Converter  PhysicalDomain=network_engine_domain  SubClassName=ps_input  LeftPortType=input  RightPortType=output  PseudoPeriodic=off  Frequencies=[]  NoiseDistribution=none  NoiseParameters=[]  Unit=1  AffineConversion=off  FilteringAndDerivatives=provide  SimscapeFilterOrder=1  InputFilterTimeConstant=0.001  UdotUserProvided=0
  Simulink-PS Converter2 : nesl_utility/Simulink-PS Converter  PhysicalDomain=network_engine_domain  SubClassName=ps_input  LeftPortType=input  RightPortType=output  PseudoPeriodic=off  Frequencies=[]  NoiseDistribution=none  NoiseParameters=[]  Unit=1  AffineConversion=off  FilteringAndDerivatives=provide  SimscapeFilterOrder=1  InputFilterTimeConstant=0.001  UdotUserProvided=0
  Skeleton : sm_lib/Body Elements/File Solid  ExtGeomFileName=C:\Users\monet\Documents\UNIVERSITA'\MAGISTRALE\Tirocinio_University_of_Poznan\MuJoco&Simscape\STL_NEW - Copia\SKELETON_COMPLETE.STL  UnitType=Custom  ExtGeomFileUnits=m  StepReaderType=HEX  ExportConvexHullGeometry=on  InertiaType=Custom  BasedOnType=Density  Density=1000  DensityUnits=kg/m^3  Mass=chassis_mass  MassUnits=kg  CenterOfMass=chassis_com  CenterOfMassUnits=m  MomentsOfInertia=chassis_I_diag  MomentsOfInertiaUnits=kg*m^2  ProductsOfInertia=chassis_I_prod  ProductsOfInertiaUnits=kg*m^2  GraphicType=FromGeometry  MarkerShape=Cube  MarkerSize=10  GraphicVisPropType=SimpleVisualProperties  GraphicDiffuseColor=[0 0.4471 0.7412]  GraphicOpacity=1  GraphicSpecularColor=[0.5 0.5 0.5 1.0]  GraphicAmbientColor=[0.15 0.15 0.15 1.0]  GraphicEmissiveColor=[0.0 0.0 0.0 1.0]  GraphicShininess=75  DoExposeReferenceFrame=on  SerializedFrames=<Frames><Frame><Id>Frame1</Id><Value><Name>F1</Name><Origin><Source>ReferenceFrame</Source><FeatureName></FeatureName></Origin><PrimaryAxis><DefinedDirection>+Z</DefinedDirection><Source>ReferenceFrame</Source><SourceDirection>+Z</SourceDirection><FeatureName></FeatureName></PrimaryAxis><SecondaryAxis><DefinedDirection>+X</DefinedDirection><Source>ReferenceFrame</Source><SourceDirection>+X</SourceDirection><FeatureName></FeatureName></SecondaryAxis></Value></Frame><Frame><Id>Frame2</Id><Value><Name>F2</Name><Origin><Source>CenterOfMassFrame</Source><FeatureName></FeatureName></Origin><PrimaryAxis><DefinedDirection>+Z</DefinedDirection><Source>ReferenceFrame</Source><SourceDirection>+Z</SourceDirection><FeatureName></FeatureName></PrimaryAxis><SecondaryAxis><DefinedDirection>+X</DefinedDirection><Source>ReferenceFrame</Source><SourceDirection>+X</SourceDirection><FeatureName></FeatureName></SecondaryAxis></Value></Frame></Frames>
  Solver Configuration : nesl_utility/Solver Configuration  PhysicalDomain=network_engine_domain  SubClassName=solver  LeftPortType=input  RightPortType=generic  Tones=[]  Harmonics=[]  SimulateNoise=off  Profile=off  UseLocalSampling=off  EnableSwitchedLinearOptims=on  FrequencyDomain=off  UseCCode=off  RelTol=0.001  AbsTol=1e-06  MinStep=1e-09  ToWorkspace=off  RevertToSquareIcSolve=off  NumHomotopyIterations=100  PhasorMode=off  PhasorModeNumHarmonics=1  ConsistencySolver=NEWTON_XTOL_AFTER_FTOL  IndexReductionMethod=DerivativeReplacement  DoDC=off  ResidualTolerance=1e-09  ConsistencyTolSource=GLOBAL  ConsistencyAbsTol=0.001  ConsistencyRelTol=0.001  ConsistencyTolFactor=0.001  UseLocalSolver=off  LocalSolverChoice=NE_BACKWARD_EULER_ADVANCER  ResolveIndetEquations=on  FunctionEvalNumThread=1  LocalSolverSampleTime=0.001  DoFixedCost=off  MaxNonlinIter=3  MaxModeIter=2  ComputeImpulses=off  ImpulseIterations=2  LinearAlgebra=Sparse  LinearAlgebraNumThread=0  EquationFormulation=NE_TIME_EF  DelaysMemoryBudget=1024  AutomaticFiltering=on  FilteringTimeConstant=0.001  PartitionStorageMethod=AS_NEEDED  PartitionMemoryBudget=1024  PartitionMethod=FAST  MultibodyUseLocalSolver=off  MultibodyLocalSolverChoice=ODE1  MultibodyLocalSolverSampleTime=0.001
  Spatial Contact Force3 : sm_lib/Forces and Torques/Spatial Contact Force  Commented=on  NormalForceType=SmoothSpringDamper  NormalStiffness=1e6  NormalStiffnessUnits=N/m  NormalDamping=1e3  NormalDampingUnits=N/(m/s)  NormalTransitionRegionWidth=1e-4  NormalTransitionRegionWidthUnits=m  FrictionType=None  CoefficientOfStaticFriction=0.5  CoefficientOfDynamicFriction=0.3  FrictionalCriticalVelocity=1e-3  FrictionalCriticalVelocityUnits=m/s  SenseContactSignal=off  SensePenetrationDepth=off  SenseSeparationDistance=off  SenseNormalForceMagnitude=off  SenseFrictionalForceMagnitude=off  SenseNormalVelocity=off  SenseTangentialVelocity=off  SenseContactBaseRotation=off  SenseContactBaseTranslation=off  SenseContactFollowerRotation=off  SenseContactFollowerTranslation=off  ZeroCrossDetectContactStartAndEnd=off
  Spatial Contact Force4 : sm_lib/Forces and Torques/Spatial Contact Force  NormalForceType=SmoothSpringDamper  NormalStiffness=1e6  NormalStiffnessUnits=N/m  NormalDamping=1e3  NormalDampingUnits=N/(m/s)  NormalTransitionRegionWidth=1e-4  NormalTransitionRegionWidthUnits=m  FrictionType=SmoothStickSlip  CoefficientOfStaticFriction=mu_static  CoefficientOfDynamicFriction=mu_kinematic  FrictionalCriticalVelocity=1e-3  FrictionalCriticalVelocityUnits=m/s  SenseContactSignal=off  SensePenetrationDepth=off  SenseSeparationDistance=on  SenseNormalForceMagnitude=on  SenseFrictionalForceMagnitude=off  SenseNormalVelocity=off  SenseTangentialVelocity=off  SenseContactBaseRotation=off  SenseContactBaseTranslation=off  SenseContactFollowerRotation=off  SenseContactFollowerTranslation=off  ZeroCrossDetectContactStartAndEnd=off
  Spatial Contact Force5 : sm_lib/Forces and Torques/Spatial Contact Force  NormalForceType=SmoothSpringDamper  NormalStiffness=1e6  NormalStiffnessUnits=N/m  NormalDamping=1e3  NormalDampingUnits=N/(m/s)  NormalTransitionRegionWidth=1e-4  NormalTransitionRegionWidthUnits=m  FrictionType=SmoothStickSlip  CoefficientOfStaticFriction=mu_static  CoefficientOfDynamicFriction=mu_kinematic  FrictionalCriticalVelocity=1e-3  FrictionalCriticalVelocityUnits=m/s  SenseContactSignal=off  SensePenetrationDepth=off  SenseSeparationDistance=on  SenseNormalForceMagnitude=on  SenseFrictionalForceMagnitude=off  SenseNormalVelocity=off  SenseTangentialVelocity=off  SenseContactBaseRotation=off  SenseContactBaseTranslation=off  SenseContactFollowerRotation=off  SenseContactFollowerTranslation=off  ZeroCrossDetectContactStartAndEnd=off
  World Frame : sm_lib/Frames and Transforms/World Frame
  Yaw pos/vel : Scope  NumInputPorts=2
  motor_torque_limits_L : Saturate  UpperLimit=motor_max_torque  LowerLimit=-motor_max_torque
  motor_torque_limits_R : Saturate  UpperLimit=motor_max_torque  LowerLimit=-motor_max_torque
  static_friction_L : DeadZone  LowerValue=-joint_friction  UpperValue=joint_friction
  static_friction_R : DeadZone  LowerValue=-joint_friction  UpperValue=joint_friction
  yaw+translations : sm_lib/Joints/Planar Joint  JointMode=Normal  CompositeWrenchDir=FollowerOnBase  CompositeWrenchFrame=BaseFrame  SenseConstraintForce=off  SenseConstraintTorque=on  SenseTotalForce=on  SenseTotalTorque=off  PxPositionTargetSpecify=off  PxPositionTargetPriority=High  PxPositionTargetValue=0  PxPositionTargetValueUnits=m  PxVelocityTargetSpecify=off  PxVelocityTargetPriority=High  PxVelocityTargetValue=0  PxVelocityTargetValueUnits=m/s  PxEquilibriumPosition=0  PxEquilibriumPositionUnits=m  PxSpringStiffness=0  PxSpringStiffnessUnits=N/m  PxDampingCoefficient=0  PxDampingCoefficientUnits=N/(m/s)  PxLowerLimitSpecify=off  PxLowerLimitBound=-1  PxLowerLimitBoundUnits=m  PxLowerLimitStiffness=1e6  PxLowerLimitStiffnessUnits=N/m  PxLowerLimitDamping=1e3  PxLowerLimitDampingUnits=N/(m/s)  PxLowerLimitTransitionRegionWidth=1e-4  PxLowerLimitTransitionRegionWidthUnits=m  PxUpperLimitSpecify=off  PxUpperLimitBound=1  PxUpperLimitBoundUnits=m  PxUpperLimitStiffness=1e6  PxUpperLimitStiffnessUnits=N/m  PxUpperLimitDamping=1e3  PxUpperLimitDampingUnits=N/(m/s)  PxUpperLimitTransitionRegionWidth=1e-4  PxUpperLimitTransitionRegionWidthUnits=m  PxTorqueActuationMode=NoTorque  PxMotionActuationMode=ComputedMotion  PxSensePosition=off  PxSenseVelocity=off  PxSenseAcceleration=off  PxSenseTorqueForce=off  PxSenseLowerLimitTorqueForce=off  PxSenseUpperLimitTorqueForce=off  PyPositionTargetSpecify=off  PyPositionTargetPriority=High  PyPositionTargetValue=0  PyPositionTargetValueUnits=m  PyVelocityTargetSpecify=off  PyVelocityTargetPriority=High  PyVelocityTargetValue=0  PyVelocityTargetValueUnits=m/s  PyEquilibriumPosition=0  PyEquilibriumPositionUnits=m  PySpringStiffness=0  PySpringStiffnessUnits=N/m  PyDampingCoefficient=0  PyDampingCoefficientUnits=N/(m/s)  PyLowerLimitSpecify=off  PyLowerLimitBound=-1  PyLowerLimitBoundUnits=m  PyLowerLimitStiffness=1e6  PyLowerLimitStiffnessUnits=N/m  PyLowerLimitDamping=1e3  PyLowerLimitDampingUnits=N/(m/s)  PyLowerLimitTransitionRegionWidth=1e-4  PyLowerLimitTransitionRegionWidthUnits=m  PyUpperLimitSpecify=off  PyUpperLimitBound=1  PyUpperLimitBoundUnits=m  PyUpperLimitStiffness=1e6  PyUpperLimitStiffnessUnits=N/m  PyUpperLimitDamping=1e3  PyUpperLimitDampingUnits=N/(m/s)  PyUpperLimitTransitionRegionWidth=1e-4  PyUpperLimitTransitionRegionWidthUnits=m  PyTorqueActuationMode=NoTorque  PyMotionActuationMode=ComputedMotion  PySensePosition=off  PySenseVelocity=off  PySenseAcceleration=off  PySenseTorqueForce=off  PySenseLowerLimitTorqueForce=off  PySenseUpperLimitTorqueForce=off  RzPositionTargetSpecify=off  RzPositionTargetPriority=High  RzPositionTargetValue=0  RzPositionTargetValueUnits=deg  RzVelocityTargetSpecify=off  RzVelocityTargetPriority=High  RzVelocityTargetValue=0  RzVelocityTargetValueUnits=deg/s  RzEquilibriumPosition=0  RzEquilibriumPositionUnits=deg  RzSpringStiffness=0  RzSpringStiffnessUnits=N*m/deg  RzDampingCoefficient=0  RzDampingCoefficientUnits=N*m/(deg/s)  RzLowerLimitSpecify=off  RzLowerLimitBound=-90  RzLowerLimitBoundUnits=deg  RzLowerLimitStiffness=1e4  RzLowerLimitStiffnessUnits=N*m/deg  RzLowerLimitDamping=10  RzLowerLimitDampingUnits=N*m/(deg/s)  RzLowerLimitTransitionRegionWidth=0.1  RzLowerLimitTransitionRegionWidthUnits=deg  RzUpperLimitSpecify=off  RzUpperLimitBound=90  RzUpperLimitBoundUnits=deg  RzUpperLimitStiffness=1e4  RzUpperLimitStiffnessUnits=N*m/deg  RzUpperLimitDamping=10  RzUpperLimitDampingUnits=N*m/(deg/s)  RzUpperLimitTransitionRegionWidth=0.1  RzUpperLimitTransitionRegionWidthUnits=deg  RzTorqueActuationMode=NoTorque  RzMotionActuationMode=ComputedMotion  RzSensePosition=on  RzSenseVelocity=on  RzSenseAcceleration=off  RzSenseTorqueForce=off  RzSenseLowerLimitTorqueForce=off  RzSenseUpperLimitTorqueForce=off
  theta_R_wheel : Outport
  theta_L_wheel : Outport  Port=2
  lin_acc : Outport  Port=3
  ang_vel : Outport  Port=4
  wires:
  PS-Simulink Converter2/1 -> lin_acc/1
  PS-Simulink Converter1/1 -> ang_vel/1
  PS-Simulink Converter3/1 -> theta_L_wheel/1
  PS-Simulink Converter/1 -> theta_R_wheel/1
  static_friction_R/1 -> motor_torque_limits_R/1
  torque_L_wheel/1 -> static_friction_L/1
  motor_torque_limits_R/1 -> Simulink-PS Converter2/1
  motor_torque_limits_L/1 -> Simulink-PS Converter1/1
  torque_R_wheel/1 -> static_friction_R/1
  static_friction_L/1 -> motor_torque_limits_L/1
  PS-Simulink Converter6/1 -> R_wheel_distance_force/1  "sep"
  PS-Simulink Converter7/1 -> R_wheel_distance_force/2  "fn"
  PS-Simulink Converter4/1 -> L_wheel_distance_force/1  "sep"
  PS-Simulink Converter5/1 -> L_wheel_distance_force/2  "fn"
  PS-Simulink Converter8/1 -> Planar_force/1  "fc"
  PS-Simulink Converter9/1 -> Planar_force/2  "ft"
  PS-Simulink Converter10/1 -> Yaw pos/vel/1  "qz"
  PS-Simulink Converter11/1 -> Yaw pos/vel/2  "wz"
  PS-Simulink Converter12/1 -> Pitch pos/vel/1  "q_pitch"
  PS-Simulink Converter13/1 -> Pitch pos/vel/2  "w_pitch"
  ext_force/1 -> Simulink-PS Converter/1
  connections:
  Ground/RConn1 -- Rigid Transform3/RConn1
  Ground/LConn1 -- Spatial Contact Force5/LConn1 -- Spatial Contact Force3/LConn1 -- Spatial Contact Force4/LConn1
  Rigid Transform5/LConn1 -- Pitch/RConn1 -- Revolute Joint2/LConn1 -- Revolute Joint1/LConn1
  World Frame/RConn1 -- Mechanism Configuration/RConn1 -- Rigid Transform12/LConn1 -- IMU/LConn1 -- Rigid Transform3/LConn1 -- Solver Configuration/RConn1
  Ghost_wheel_L/RConn1 -- Spatial Contact Force4/RConn1
  Rigid Transform/RConn1 -- Skeleton/RConn1
  Simulink-PS Converter1/RConn1 -- Revolute Joint1/LConn2
  Rigid Transform6/LConn1 -- Rigid Transform2/LConn1 -- Motor_Inertia_L/RConn1 -- Revolute Joint1/RConn1
  IMU/RConn2 -- PS-Simulink Converter1/LConn1
  Rigid Transform6/RConn1 -- Ghost_wheel_L/LConn1
  IMU/RConn1 -- Rigid Transform/LConn1
  PS-Simulink Converter2/LConn1 -- IMU/RConn3
  Revolute Joint2/RConn2 -- PS-Simulink Converter/LConn1
  Revolute Joint2/RConn1 -- Rigid Transform1/LConn1 -- Rigid Transform7/LConn1 -- Motor_Inertia_R/RConn1
  Spatial Contact Force5/RConn1 -- Ghost_wheel_R/RConn1
  Skeleton/RConn2 -- Spatial Contact Force3/RConn1
  Revolute Joint1/RConn2 -- PS-Simulink Converter3/LConn1
  Simulink-PS Converter2/RConn1 -- Revolute Joint2/LConn2
  Rigid Transform7/RConn1 -- R_wheel/LConn1
  Rigid Transform1/RConn1 -- Ghost_wheel_R/LConn1
  Rigid Transform2/RConn1 -- L_wheel/LConn1
  Skeleton/LConn1 -- Rigid Transform5/RConn1
  Spatial Contact Force4/RConn2 -- PS-Simulink Converter4/LConn1
  PS-Simulink Converter5/LConn1 -- Spatial Contact Force4/RConn3
  PS-Simulink Converter7/LConn1 -- Spatial Contact Force5/RConn3
  Spatial Contact Force5/RConn2 -- PS-Simulink Converter6/LConn1
  yaw+translations/RConn5 -- PS-Simulink Converter9/LConn1
  yaw+translations/RConn1 -- Rigid Transform13/LConn1
  Rigid Transform14/RConn1 -- Pitch/LConn1
  yaw+translations/LConn1 -- Rigid Transform12/RConn1
  yaw+translations/RConn4 -- PS-Simulink Converter8/LConn1
  Rigid Transform13/RConn1 -- Rigid Transform14/LConn1
  yaw+translations/RConn2 -- PS-Simulink Converter10/LConn1
  yaw+translations/RConn3 -- PS-Simulink Converter11/LConn1
  Pitch/RConn2 -- PS-Simulink Converter12/LConn1
  Pitch/RConn3 -- PS-Simulink Converter13/LConn1
  External Force and Torque/RConn1 -- Skeleton/LConn2
  Simulink-PS Converter/RConn1 -- External Force and Torque/LConn1

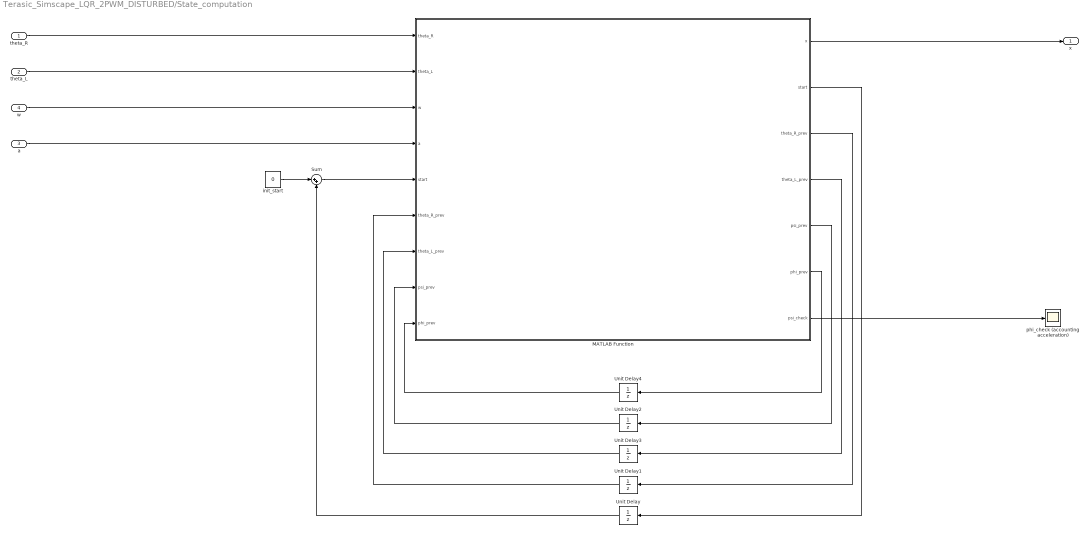
== system Terasic_Simscape_LQR_2PWM_DISTURBED/State_computation ==
  theta_R : Inport
  theta_L : Inport  Port=2
  a : Inport  Port=3
  w : Inport  Port=4
  MATLAB Function : MATLAB Function  TreatAsAtomicUnit=on
  Sum : Sum  Inputs=|++
  Unit Delay{,1..4} (5 alike) : UnitDelay  SampleTime=dt  HasFrameUpgradeWarning=on
  init_start : Constant  Value=0
  phi_check (accounting acceleration) : Scope
  x : Outport
  wires:
  theta_L/1 -> MATLAB Function/2(theta_L)
  MATLAB Function/3(theta_R_prev) -> Unit Delay1/1
  Unit Delay1/1 -> MATLAB Function/6("theta_R_prev ")
  theta_R/1 -> MATLAB Function/1(theta_R)
  Unit Delay/1 -> Sum/2
  MATLAB Function/4(theta_L_prev) -> Unit Delay3/1
  Unit Delay3/1 -> MATLAB Function/7("theta_L_prev ")
  MATLAB Function/2(start) -> Unit Delay/1
  init_start/1 -> Sum/1
  Sum/1 -> MATLAB Function/5("start ")
  MATLAB Function/1(x) -> x/1
  w/1 -> MATLAB Function/3(w)
  a/1 -> MATLAB Function/4(a)
  MATLAB Function/5(psi_prev) -> Unit Delay2/1
  Unit Delay2/1 -> MATLAB Function/8("psi_prev ")
  MATLAB Function/6(phi_prev) -> Unit Delay4/1
  Unit Delay4/1 -> MATLAB Function/9("phi_prev ")
  MATLAB Function/7(psi_check) -> phi_check (accounting acceleration)/1

== matlab function Terasic_Simscape_LQR_2PWM_DISTURBED/State_computation/MATLAB Function ==
  data: theta_R input; x output; theta_L input; w input; a input; start input; theta_R_prev input; theta_L_prev input; wheel_radius parameter; wheel_track parameter; dt parameter; psi_prev input; start output; theta_R_prev output; theta_L_prev output; psi_prev output; phi_prev input; phi_prev output; psi_check output
function [x, start, theta_R_prev, theta_L_prev, psi_prev, phi_prev, psi_check] = ...
    state_estimator(theta_R, theta_L, w, a, ...
                    start, theta_R_prev, theta_L_prev, wheel_radius, wheel_track, dt, psi_prev, phi_prev)
psi_check = 0;
% STATE_ESTIMATOR
% Vettore di stato:
%   x = [theta; psi; phi; theta_dot; psi_dot; phi_dot]
%
% theta_R, theta_L : angoli encoder delle ruote [rad]
% psi        : posizione del giunto di pitch [rad]
% psi_dot   : velocità del giunto di pitch [rad/s]
% start            : flag di inizializzazione
% theta_R_prev,
% theta_L_prev     : angoli delle ruote al campione precedente [rad]
% wheel_radius     : raggio ruota [m]
% wheel_track      : distanza tra le ruote [m]
% dt               : intervallo di campionamento [s]


    % Protezione da parametri non validi
    if dt <= 0 || wheel_track == 0
        x = zeros(6,1);
        return;
    end

    % Inizializza le memorie degli encoder senza generare un picco
    % artificiale di velocità al primo campione.
    if start == 0
        theta_R_prev = theta_R;
        theta_L_prev = theta_L;
        psi_prev = 0;
        phi_prev = 0;
        start = 1;
    end

    % Velocità angolari delle ruote da differenza discreta
    theta_R_dot = (theta_R - theta_R_prev) / dt;
    theta_L_dot = (theta_L - theta_L_prev) / dt;

    % Aggiorna le memorie per il campione successivo
    theta_R_prev = theta_R;
    theta_L_prev = theta_L;

    % Pitch_dot ottenuto dall'IMU
    psi_dot = -w(1);  % it's the pitch_dot detected

    % Pitch computation
    %%% IT NEEDS KALMAN FILTER FOR THE NOISE, BUT IT'S MORE ACCURATE
    %%% ACCOUNTING THE ACCELERATION
    psi_acc = -atan2(a(3), a(1));

    alpha = 0.99;
    psi_comp = alpha * (psi_prev + psi_dot * dt) ...
        + (1 - alpha) * psi_acc;
    psi_check = psi_comp;
    
    psi = psi_prev + psi_dot * dt;

    psi_prev = psi;


    % Rotazione media delle ruote
    theta_enc_mean = (theta_R + theta_L) / 2;
    theta_enc_dot  = (theta_R_dot + theta_L_dot) / 2;

    theta     = theta_enc_mean + psi;
    theta_dot = theta_enc_dot  + psi_dot;

    % Yaw ricavato dalla IMU
    % phi = (wheel_radius / wheel_track) * (theta_R - theta_L);
    % phi_dot = (wheel_radius / wheel_track) * ...
    %           (theta_R_dot - theta_L_dot);
    phi_dot = -w(3);
    phi = phi_prev + phi_dot * dt;
    phi_prev = phi;

    % Ordine richiesto dal controllore
    x = [theta;
         psi;
         phi;
         theta_dot;
         psi_dot;
         phi_dot];
end
